simulink model "dc_fed_grid_connected_vsi_open_loop_simscape2026"  (R2026a)
settings: Solver=ode23t  StopTime=0.1  FixedStep=1e-5
undefined symbols (not defined in the file): Three_PhaseSource_class, Three_PhaseV_IMeasuremen_class, UniversalBridge_class
libraries: nesl_utility x10, ee_lib x5, fl_lib x3, eePwmGeneratorTwoLevel x1
settings Model: Creator=HAKAN SARI  LastModifiedBy=HAKAN SARI
settings DebuggingCC: SaveWithParameterizedLinksMsg=none
settings SimscapeCC: SimscapeLogType=none  SimscapeLogDataHistory=5000.0

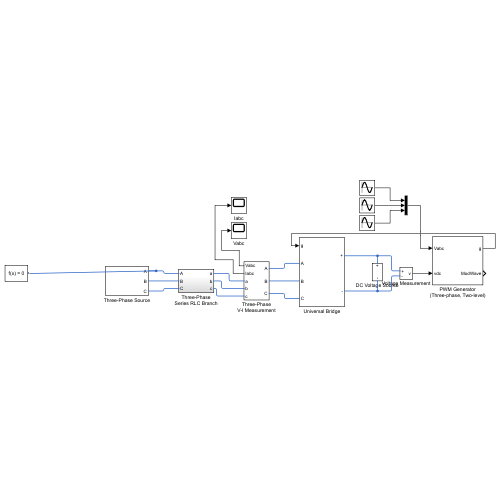
[thumbnail: Simulink's stored preview of the top-level diagram]
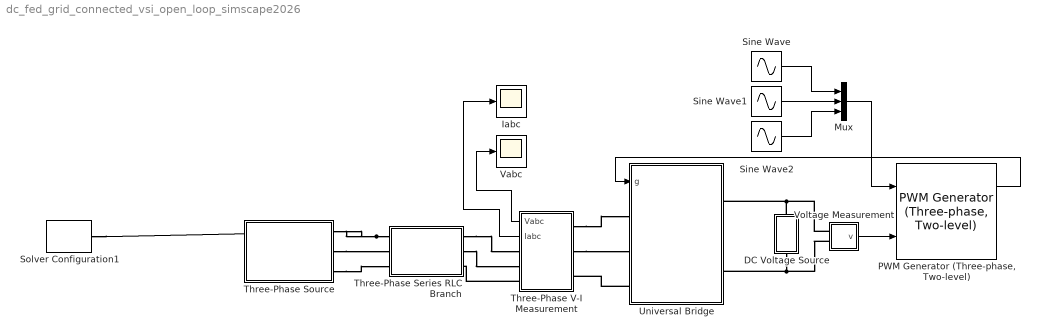
== system dc_fed_grid_connected_vsi_open_loop_simscape2026 ==
  DC Voltage Source : Subsystem
      settings: OpenFcn=elec.conv.unmask(gcb);
  Iabc : Scope
      settings: ActiveDisplayYMinimum=-0.0081648678196405387  ActiveDisplayYMaximum=0.0081648678196408683
  Mux : Mux  Inputs=3
  "PWM Generator (Three-phase, Two-level)" : eePwmGeneratorTwoLevel/PWM Generator (Three-phase, Two-level)  PWMMode=Continuous PWM (CPWM)  CPWMMode=SPWM: sinusoidal PWM  DPWMMode=60 DPWM: 60 degree discontinuous PWM  fsw=5e3  Ts=1e-5
      settings: LibrarySourceBlock=|
      | ee_sl_lib/Pulse Width
      | Modulation/PWM Generator
      | (Three-phase, Two-level)
  Sine Wave : Sin  Amplitude=0.5  Frequency=314.159  SampleTime=0
  Sine Wave1 : Sin  Amplitude=0.5  Frequency=314.159  Phase=-2*pi/3  SampleTime=0
  Sine Wave2 : Sin  Amplitude=0.5  Frequency=314.159  Phase=2*pi/3  SampleTime=0
  Solver Configuration1 : nesl_utility/Solver Configuration  PhysicalDomain=network_engine_domain  SubClassName=solver  LeftPortType=input  RightPortType=generic  Tones=[]  Harmonics=[]  SimulateNoise=off  Profile=off  UseLocalSampling=off  EnableSwitchedLinearOptims=on  FrequencyDomain=off  UseCCode=off  RelTol=0.001  AbsTol=0.001  MinStep=1e-09  ToWorkspace=off  RevertToSquareIcSolve=off  NumHomotopyIterations=100  PhasorMode=off  PhasorModeNumHarmonics=1  ConsistencySolver=NEWTON_XTOL_AFTER_FTOL  CanonicalOrdering=CANONICAL  OptimizeIntermediates=OPTIMIZED  IndexReductionMethod=DerivativeReplacement  DoDC=off  ResidualTolerance=1e-09  ConsistencyTolSource=GLOBAL  ConsistencyAbsTol=0.001  ConsistencyRelTol=0.001  ConsistencyTolFactor=0.001  UseLocalSolver=off  LocalSolverChoice=NE_BACKWARD_EULER_ADVANCER  ResolveIndetEquations=on  FunctionEvalNumThread=1  LocalSolverSampleTime=0.001  DoFixedCost=off  MaxNonlinIter=3  MaxModeIter=2  ComputeImpulses=off  ImpulseIterations=2  LinearAlgebra=auto  LinearAlgebraNumThread=0  EquationFormulation=NE_TIME_EF  DelaysMemoryBudget=1024  AutomaticFiltering=on  FilteringTimeConstant=0.001  PartitionStorageMethod=AS_NEEDED  PartitionMemoryBudget=1024  PartitionMethod=ROBUST  MultibodyUseLocalSolver=off  MultibodyLocalSolverChoice=ODE1  MultibodyLocalSolverSampleTime=0.001
  Three-Phase Series RLC Branch : Subsystem
      settings: AttributesFormatString=\n
  Three-Phase V-I Measurement : Subsystem
      settings: OpenFcn=elec.conv.unmask(gcb);
  Three-Phase Source : Subsystem
      settings: OpenFcn=elec.conv.unmask(gcb);
  Universal Bridge : Subsystem
      settings: OpenFcn=elec.conv.unmask(gcb);
  Vabc : Scope
      settings: ActiveDisplayYMinimum=-408.24339098200716  ActiveDisplayYMaximum=408.24339098202279
  Voltage Measurement : Subsystem
      settings: OpenFcn=elec.conv.unmask(gcb);
  wires:
  Voltage Measurement/1(v) -> "PWM Generator (Three-phase, Two-level)"/2
  Sine Wave/1 -> Mux/1
  Sine Wave1/1 -> Mux/2
  Sine Wave2/1 -> Mux/3
  Mux/1 -> "PWM Generator (Three-phase, Two-level)"/1
  "PWM Generator (Three-phase, Two-level)"/1 -> Universal Bridge/1(g)
  Three-Phase V-I Measurement/1(Vabc) -> Vabc/1
  Three-Phase V-I Measurement/2(Iabc) -> Iabc/1
  connections:
  DC Voltage Source/RConn1 -- Voltage Measurement/LConn1 -- Universal Bridge/RConn1
  DC Voltage Source/LConn1 -- Voltage Measurement/LConn2 -- Universal Bridge/RConn2
  Three-Phase Series RLC Branch/LConn1 -- Three-Phase Source/RConn1 -- Solver Configuration1/RConn1
  Three-Phase Source/RConn2 -- Three-Phase Series RLC Branch/LConn2
  Three-Phase Source/RConn3 -- Three-Phase Series RLC Branch/LConn3
  Three-Phase Series RLC Branch/RConn1 -- Three-Phase V-I Measurement/RConn1
  Three-Phase Series RLC Branch/RConn2 -- Three-Phase V-I Measurement/RConn2
  Three-Phase V-I Measurement/RConn3 -- Three-Phase Series RLC Branch/RConn3
  Three-Phase V-I Measurement/LConn1 -- Universal Bridge/LConn1
  Three-Phase V-I Measurement/LConn2 -- Universal Bridge/LConn2
  Universal Bridge/LConn3 -- Three-Phase V-I Measurement/LConn3

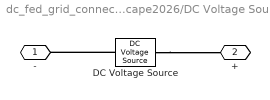
== system dc_fed_grid_connected_vsi_open_loop_simscape2026/DC Voltage Source ==
  DC Voltage Source : fl_lib/Electrical/Electrical Sources/DC Voltage Source  v0=700 V
  - : PMIOPort  Side=Left
  + : PMIOPort  Port=2  Side=Right
  connections:
  DC Voltage Source/RConn1 -- -/RConn1
  DC Voltage Source/LConn1 -- +/RConn1

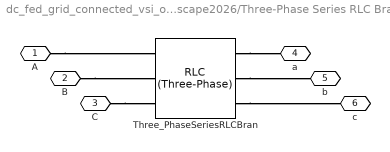
== system dc_fed_grid_connected_vsi_open_loop_simscape2026/Three-Phase Series RLC Branch ==
  Three_PhaseSeriesRLCBran : ee_lib/Passive/RLC Assemblies/RLC (Three-Phase)  port_option=ee.enum.threePhasePort.expanded  component_structure=7  R=0.5 Ohm  L=0.005 H  C=0.0000001 F  R_parasitic=1e-6 Ohm  G_parasitic=1e-6 1/Ohm  IL_specify=on  IL_priority=High  IL=[0, 0, 0] A  IL_nominal_specify=off  IL_nominal_value=1  IL_nominal_unit=A  VC_specify=on  VC_priority=High  VC=[0, 0, 0] V  VC_nominal_specify=off  VC_nominal_value=1  VC_nominal_unit=V
  A : PMIOPort  Side=Left
  B : PMIOPort  Port=2  Side=Left
  C : PMIOPort  Port=3  Side=Left
  a : PMIOPort  Port=4  Side=Right
  b : PMIOPort  Port=5  Side=Right
  c : PMIOPort  Port=6  Side=Right
  connections:
  Three_PhaseSeriesRLCBran/RConn3 -- c/RConn1
  Three_PhaseSeriesRLCBran/RConn2 -- b/RConn1
  Three_PhaseSeriesRLCBran/RConn1 -- a/RConn1
  C/RConn1 -- Three_PhaseSeriesRLCBran/LConn3
  B/RConn1 -- Three_PhaseSeriesRLCBran/LConn2
  A/RConn1 -- Three_PhaseSeriesRLCBran/LConn1

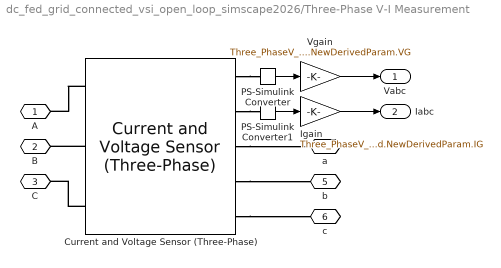
== system dc_fed_grid_connected_vsi_open_loop_simscape2026/Three-Phase V-I Measurement ==
  Current and Voltage Sensor (Three-Phase) : ee_lib/Sensors & Transducers/Current and Voltage Sensor (Three-Phase)  port_option=ee.enum.threePhasePort.expanded  vMeasurementType=2  outputUnit=2  SRated=100000000 V*A  VRated=500000 V  I_specify=off  I_priority=None  I=[ 0 0 0 ] A  I_nominal_specify=off  I_nominal_value=1  I_nominal_unit=A  V_specify=off  V_priority=None  V=[ 0 0 0 ] V  V_nominal_specify=off  V_nominal_value=1  V_nominal_unit=V
  Igain : Gain  Gain=Three_PhaseV_IMeasuremen_class('phase-to-ground','yes','off','off','off',100000000,500000).objParamMappingDerived.NewDerivedParam.IG
  PS-Simulink Converter : nesl_utility/PS-Simulink Converter  PhysicalDomain=network_engine_domain  SubClassName=ps_output  LeftPortType=input  RightPortType=output  PseudoPeriodic=off  Frequencies=[]  VectorFormat=1-D array  Unit=1  AffineConversion=off
  PS-Simulink Converter1 : nesl_utility/PS-Simulink Converter  PhysicalDomain=network_engine_domain  SubClassName=ps_output  LeftPortType=input  RightPortType=output  PseudoPeriodic=off  Frequencies=[]  VectorFormat=1-D array  Unit=1  AffineConversion=off
  Vgain : Gain  Gain=Three_PhaseV_IMeasuremen_class('phase-to-ground','yes','off','off','off',100000000,500000).objParamMappingDerived.NewDerivedParam.VG
  A : PMIOPort  Side=Left
  B : PMIOPort  Port=2  Side=Left
  C : PMIOPort  Port=3  Side=Left
  a : PMIOPort  Port=4  Side=Right
  b : PMIOPort  Port=5  Side=Right
  c : PMIOPort  Port=6  Side=Right
  Vabc : Outport  VectorParamsAs1DForOutWhenUnconnected=off
  Iabc : Outport  Port=2  VectorParamsAs1DForOutWhenUnconnected=off
  wires:
  Igain/1 -> Iabc/1
  Vgain/1 -> Vabc/1
  PS-Simulink Converter1/1 -> Igain/1
  PS-Simulink Converter/1 -> Vgain/1
  connections:
  Current and Voltage Sensor (Three-Phase)/RConn1 -- PS-Simulink Converter/LConn1
  Current and Voltage Sensor (Three-Phase)/RConn2 -- PS-Simulink Converter1/LConn1
  Current and Voltage Sensor (Three-Phase)/RConn5 -- c/RConn1
  Current and Voltage Sensor (Three-Phase)/RConn4 -- b/RConn1
  Current and Voltage Sensor (Three-Phase)/RConn3 -- a/RConn1
  Current and Voltage Sensor (Three-Phase)/LConn3 -- C/RConn1
  Current and Voltage Sensor (Three-Phase)/LConn1 -- A/RConn1
  Current and Voltage Sensor (Three-Phase)/LConn2 -- B/RConn1

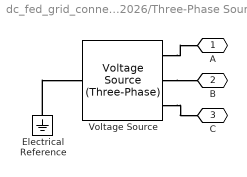
== system dc_fed_grid_connected_vsi_open_loop_simscape2026/Three-Phase Source ==
  Electrical Reference : fl_lib/Electrical/Electrical Elements/Electrical Reference
  Voltage Source : ee_lib/Sources/Voltage Source (Three-Phase)  vline_rms=400 V  shift=0 deg  freq=50 Hz  impedance_option=4  SShortCircuit=100000000 V*A  XR=7  R=Three_PhaseSource_class(400,50,0.1,0.001,100000000,400,7,'on','off').objParamMappingDerived.NewDerivedParam.R Ohm  L=Three_PhaseSource_class(400,50,0.1,0.001,100000000,400,7,'on','off').objParamMappingDerived.NewDerivedParam.L H  harmonic_option=0  harmonic_orders=[5, 7, 11, 13]  harmonic_ratios=[.1, .1, .1, .1]  G_parasitic=0 1/Ohm  I_specify=off  I_priority=None  I=[ 0 0 0 ] A  I_nominal_specify=off  I_nominal_value=1  I_nominal_unit=A
  A : PMIOPort  Side=Right
  B : PMIOPort  Port=2  Side=Right
  C : PMIOPort  Port=3  Side=Right
  connections:
  Voltage Source/RConn2 -- B/RConn1
  Voltage Source/RConn1 -- A/RConn1
  Voltage Source/RConn3 -- C/RConn1
  Electrical Reference/LConn1 -- Voltage Source/LConn1

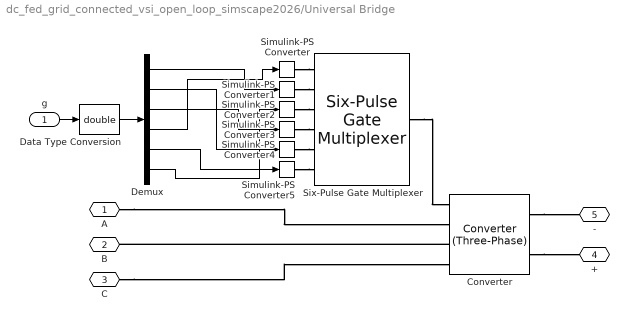
== system dc_fed_grid_connected_vsi_open_loop_simscape2026/Universal Bridge ==
  g : Inport
  Converter : ee_lib/Semiconductors & Converters/Converters/Converter (Three-Phase)  port_option=ee.enum.threePhasePort.expanded  fidelity_option=ee.enum.converters.fidelity.detailed  device_type=ee.enum.converters.switchingdevice.thyristor  showThermalPort=false  K=0  Vth=1e-3 V  Vgt=1e-3 V  Vgt_off=-1 V  Ih=0.1 A  Vf=UniversalBridge_class('3','Thyristors',[0 0],0,100000,Inf,0.001).objParamMappingDerived.NewDerivedParam.Vf V  Ron=UniversalBridge_class('3','Thyristors',[0 0],0,100000,Inf,0.001).objParamMappingDerived.NewDerivedParam.Ron Ohm  Rds=0.001 Ohm  Goff=UniversalBridge_class('3','Thyristors',[0 0],0,100000,Inf,0.001).objParamMappingDerived.NewDerivedParam.Goff 1/Ohm  Eon_scalar=22.86e-3 J  Eoff_scalar=17.14e-3 J  Eoff_natural_commutation=10e-3 J  Voff=300 V  Iout_scalar=600 A  onCurrentMeasDelay=0 s  useCurrentFromPreviousCycle=false  useVoltageFromPreviousCycle=false  diode_param=ee.enum.converters.protectiondiode.none  diode_Vf=0.8 V  diode_Ron=0.001 Ohm  diode_Goff=1e-5 1/Ohm  diode_C=50 nF  diode_iRM=-235 A  diode_iF=300 A  diode_idot=-50 A/us  diode_trr_param=ee.enum.converters.diodetrr.trr_factor  diode_trr_factor=3  diode_trr=15 us  diode_Qrr=1.5e+3 s*uA  diode_rec_loss_model=ee.enum.diode.reverseRecoveryModel.fixed  diode_ErecVal=0 J  diode_scaleWithIandV=false  diode_ErecMat=zeros(2, 3) J  diode_TjrecVec=[298.15, 398.15] K  diode_IfrecVec=[.1, 1, 10] A  diode_IrecVal=10 A  diode_VrecVal=10 V  diode_tFilter=1 / 1000 / 100 s  thermal_network_parameterization=ee.enum.thermalNetworkTopology.external  Rth=[.08, .5] K/W  Rth_Cauer=[.08, .1, .5] K/W  Rth_Foster=[.08, .14, .22, .16] K/W  thermal_mass_parameterization=ee.enum.thermalNetwork.timeconstant  thermal_mass=[.01, .5] J/K  thermal_mass_Cauer=[.01, .1, .5] J/K  thermal_mass_Foster=[.001, .005, .05, .5] J/K  thermal_time_constant=[.001, .2] s  thermal_time_constant_Cauer=[.001, .1, .2] s  thermal_time_constant_Foster=[7e-05, .0007, .01, .08] s  thermal_mass_initial_temperatures=[25, 25] degC  thermal_mass_initial_temperatures_Cauer=[25, 25, 25] degC  junction_thermal_mass=0.01 J/K  Tvec_initial_Foster=[25, 25, 25, 25] degC  snubber_type=0  Cs=UniversalBridge_class('3','Thyristors',[0 0],0,100000,Inf,0.001).objParamMappingDerived.NewDerivedParam.Cs F  Rs=UniversalBridge_class('3','Thyristors',[0 0],0,100000,Inf,0.001).objParamMappingDerived.NewDerivedParam.Rs Ohm  Vce_loss=[0, 150, 300] V
  Data Type Conversion : DataTypeConversion  OutDataTypeStr=double  SaturateOnIntegerOverflow=off  RndMeth=Floor
  Demux : Demux  Outputs=6
  Simulink-PS Converter{,1..5} (6 alike) : nesl_utility/Simulink-PS Converter  PhysicalDomain=network_engine_domain  SubClassName=ps_input  LeftPortType=input  RightPortType=output  PseudoPeriodic=off  Frequencies=[]  NoiseDistribution=none  NoiseParameters=[]  Unit=1  AffineConversion=off  FilteringAndDerivatives=provide  SimscapeFilterOrder=1  InputFilterTimeConstant=0.001  UdotUserProvided=0
  Six-Pulse Gate Multiplexer : ee_lib/Semiconductors & Converters/Converters/Six-Pulse Gate Multiplexer  port_option=ee.enum.controlport.ps
  A : PMIOPort  Side=Left
  B : PMIOPort  Port=2  Side=Left
  C : PMIOPort  Port=3  Side=Left
  + : PMIOPort  Port=4  Side=Right
  - : PMIOPort  Port=5  Side=Right
  wires:
  Demux/6 -> Simulink-PS Converter2/1
  Demux/5 -> Simulink-PS Converter5/1
  Demux/4 -> Simulink-PS Converter/1
  Demux/3 -> Simulink-PS Converter3/1
  Demux/2 -> Simulink-PS Converter4/1
  Demux/1 -> Simulink-PS Converter1/1
  g/1 -> Data Type Conversion/1
  Data Type Conversion/1 -> Demux/1
  connections:
  Converter/RConn1 -- -/RConn1
  Converter/RConn2 -- +/RConn1
  Six-Pulse Gate Multiplexer/RConn1 -- Converter/LConn1
  Simulink-PS Converter1/RConn1 -- Six-Pulse Gate Multiplexer/LConn2
  Simulink-PS Converter/RConn1 -- Six-Pulse Gate Multiplexer/LConn1
  Simulink-PS Converter2/RConn1 -- Six-Pulse Gate Multiplexer/LConn3
  Simulink-PS Converter3/RConn1 -- Six-Pulse Gate Multiplexer/LConn4
  Simulink-PS Converter4/RConn1 -- Six-Pulse Gate Multiplexer/LConn5
  Simulink-PS Converter5/RConn1 -- Six-Pulse Gate Multiplexer/LConn6
  Converter/LConn3 -- B/RConn1
  A/RConn1 -- Converter/LConn2
  C/RConn1 -- Converter/LConn4

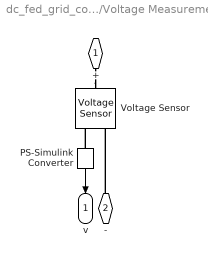
== system dc_fed_grid_connected_vsi_open_loop_simscape2026/Voltage Measurement ==
  PS-Simulink Converter : nesl_utility/PS-Simulink Converter  PhysicalDomain=network_engine_domain  SubClassName=ps_output  LeftPortType=input  RightPortType=output  PseudoPeriodic=off  Frequencies=[]  VectorFormat=1-D array  Unit=V  AffineConversion=off
  Voltage Sensor : fl_lib/Electrical/Electrical Sensors/Voltage Sensor
  + : PMIOPort  Side=Left
  - : PMIOPort  Port=2  Side=Left
  v : Outport  VectorParamsAs1DForOutWhenUnconnected=off
  wires:
  PS-Simulink Converter/1 -> v/1
  connections:
  PS-Simulink Converter/LConn1 -- Voltage Sensor/RConn1
  -/RConn1 -- Voltage Sensor/RConn2
  +/RConn1 -- Voltage Sensor/LConn1
